simulink model "b0_caller"  (R2023b)
settings: Solver=FixedStepDiscrete  StartTime=0.0  StopTime=12  FixedStep=0.001  RelTol=1e-3
settings Model: Creator=28447  LastModifiedBy=28447
settings SFSimCC: SimCustomHeaderCode=extern void b0_ident_sim(float iq, float u, float omega, float e1, float v, float *b0, float *du);  SimUserIncludeDirs=D:\Desktop\RCESO\simulink
settings SFSimCC: SimUserSources=|
  | D:\Desktop\RCESO\simulink\b0_ident.c
  | D:\Desktop\RCESO\simulink\b0_ident_wrap.c

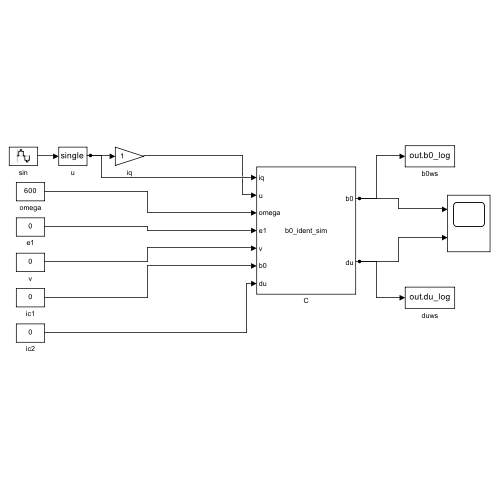
[thumbnail: Simulink's stored preview of the top-level diagram]
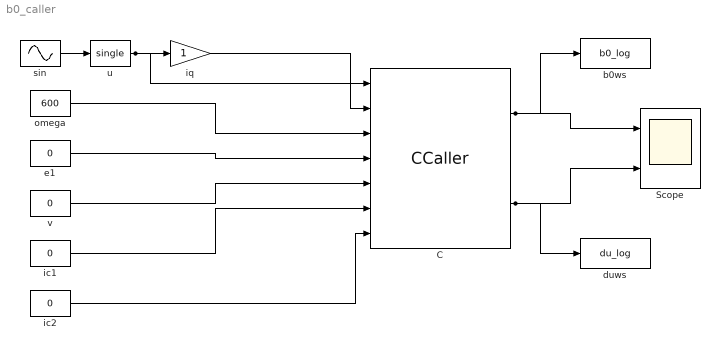
== system b0_caller ==
  C : CCaller  FunctionName=b0_ident_sim  PortSpecificationStruct="%)30     .    ^ L   8    (     @         %    \"     <    !     0         %  0 \"0    $    _    07)G3F%M90  4&]R=$YA;64 4V-O<&4     26YD97@     5'EP90      4VEZ90      27-';&]B86P   X    P    !@    @    $          4    (     0    (    !         !   @!I<0  #@   #     &    \"     0         !0    @    !     @    $         $  \" &EQ   .    .     8    (    !          %    \"     $    %     0         0  ...(+3754 chars)"
  Scope : Scope  NumInputPorts=2
  b0ws : ToWorkspace  VariableName=b0_log  SaveFormat=Timeseries  SampleTime=0.001
  duws : ToWorkspace  VariableName=du_log  SaveFormat=Timeseries  SampleTime=0.001
  e1 : Constant  Value=0  OutDataTypeStr=single  SampleTime=0.001
  ic1 : Constant  Value=0  OutDataTypeStr=single  SampleTime=0.001
  ic2 : Constant  Value=0  OutDataTypeStr=single  SampleTime=0.001
  iq : Gain  OutDataTypeStr=single
  omega : Constant  Value=600  OutDataTypeStr=single  SampleTime=0.001
  sin : Sin  Amplitude=0.118  Frequency=2*pi*65  SampleTime=0.001
  u : DataTypeConversion  OutDataTypeStr=single  SaturateOnIntegerOverflow=off  RndMeth=Floor
  v : Constant  Value=0  OutDataTypeStr=single  SampleTime=0.001
  wires:
  sin/1 -> u/1
  u/1 -> iq/1, C/1
  iq/1 -> C/2
  omega/1 -> C/3
  e1/1 -> C/4
  v/1 -> C/5
  ic1/1 -> C/6
  ic2/1 -> C/7
  C/1 -> Scope/1, b0ws/1
  C/2 -> Scope/2, duws/1
